simulink model "ArbBt"  (R2026a)
settings: Solver=FixedStepDiscrete  StopTime=10  FixedStep=0.005  EnableMultiTasking=on
undefined symbols (not defined in the file): absS, ArbBt_GradientInactive, ArbBt_GradientMax, ArbBt_GradientMin, ArbBt_PressureInactive, ArbBt_PressureMax, ArbBt_PressureMin, arbD, CLIP_HIGH_G, CLIP_HIGH_P, CLIP_LOW_G, CLIP_LOW_P, hps, ibBhms, PBP_CycleIndexTable, PBP_MAX_PROFILES, PBP_ProfileLength, PBP_ProfileStart, PBP_ProfileTable, PBP_SafeRow, PBP_StateType, ssm, tc, ysc
libraries: simulink x1
(part 1 of 2)
settings Model: DataDictionary=ArbBt_DataDictionary.sldd  Creator=72878  LastModifiedBy=72878
settings OptimizationCC: UseDivisionForNetSlopeComputation=on  DefaultUnderspecifiedDataType=single  InlineInvariantSignals=on  EfficientFloat2IntCast=on
settings DebuggingCC: SignalInfNanChecking=error  SignalRangeChecking=error  ReadBeforeWriteMsg=EnableAllAsWarning  WriteAfterWriteMsg=EnableAllAsWarning  WriteAfterReadMsg=EnableAllAsWarning  AlgebraicLoopMsg=error  ArtificialAlgebraicLoopMsg=error  SaveWithDisabledLinksMsg=error  SaveWithParameterizedLinksMsg=error  BlockPriorityViolationMsg=error  SolverPrmCheckMsg=error  InheritedTsInSrcMsg=error  MultiTaskRateTransMsg=warning  TasksWithSamePriorityMsg=error  SigSpecEnsureSampleTimeMsg=error  CheckMatrixSingularityMsg=error  IntegerOverflowMsg=error  ParameterUnderflowMsg=error  ParameterPrecisionLossMsg=error  UnderSpecifiedDataTypeMsg=error  UnnecessaryDatatypeConvMsg=warning  VectorMatrixConversionMsg=error  SignalLabelMismatchMsg=error  UnconnectedInputMsg=error  UnconnectedOutputMsg=error  UnconnectedLineMsg=error  SFcnCompatibilityMsg=error  BusObjectLabelMismatch=error  RootOutportRequireBusObject=error  AssertControl=DisableAll  ModelReferenceIOMismatchMessage=error  UnknownTsInhSupMsg=error  ModelReferenceDataLoggingMessage=error  StrictBusMsg=ErrorOnBusTreatedAsVector  NonBusSignalsTreatedAsBus=error  SFInvalidInputDataAccessInChartInitDiag=error  SFTransitionOutsideNaturalParentDiag=error  SFUnreachableExecutionPathDiag=error  SFUndirectedBroadcastEventsDiag=error  SFTransitionActionBeforeConditionDiag=error  SFTemporalDelaySmallerThanSampleTimeDiag=error  SFSelfTransitionDiag=error  SFExecutionAtInitializationDiag=error  IntegerSaturationMsg=error  VariantConditionMismatch=warning
settings SFSimCC: CompileTimeRecursionLimit=0.0  EnableRuntimeRecursion=off
settings RTWCC: SystemTargetFile=ert.tlc  EmbeddedCoderDictionary=ArbBt_DataDictionary.sldd  CustomHeaderCode="#include \"PBP_Config.h\""  CustomInclude="\"F:\\Onedrive_GN\\OneDrive - Brakes India Private Limited\\72878\\Nandini\\Electronic Stability Control\\POC\\MATLAB Models\\ARB_BT-PBP\\config\""  Description=Embedded Coder
settings CodeAppCC: IgnoreTestpoints=on  MATLABFcnDesc=on  MangleLength=4.0  MATLABSourceComments=on  ReqsInCode=on
settings ERTTargetCC: PreserveExpressionOrder=on  EnableSignedLeftShifts=off  EnableSignedRightShifts=off  UtilityFuncGeneration=Shared location  GenerateSampleERTMain=on  IncludeMdlTerminateFcn=off  SuppressErrorStatus=on  SupportNonFinite=off  ParenthesesLevel=Standards  CastingMode=Standards  GenerateSharedConstants=off
settings ConfigComp: CovScope=ReferencedModels  CovIncludeTopModel=off  CovForceBlockReductionOff=off

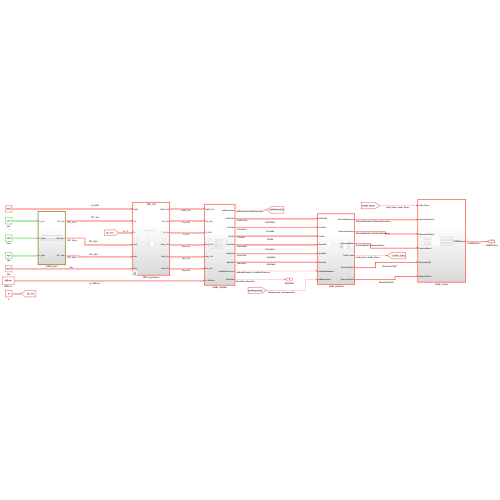
[thumbnail: Simulink's stored preview of the top-level diagram]
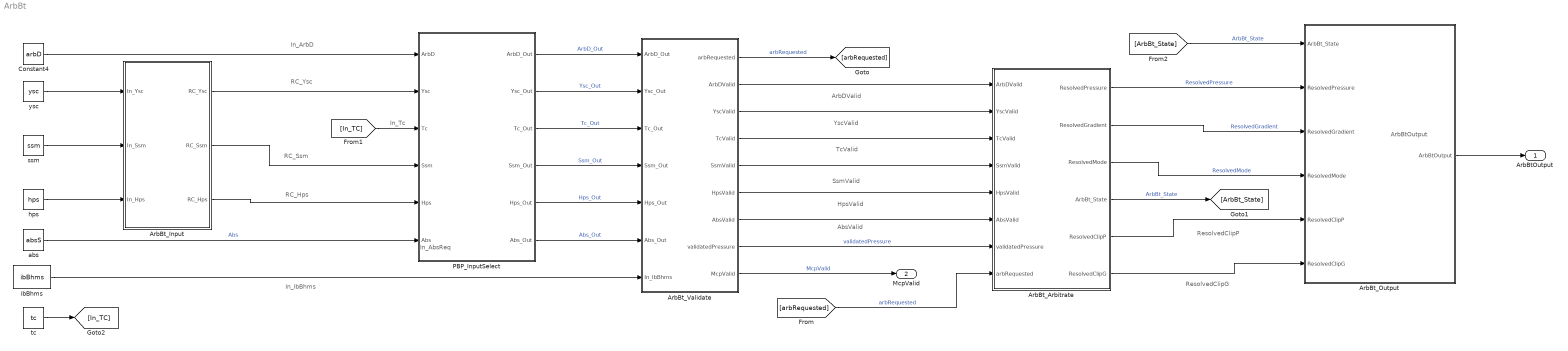
== system ArbBt ==
  note: SsmValid
  note: YscValid
  note: RC_Hps
  note: RC_Ssm
  note: RC_Ysc
  note: ArbBtOutput
  note: ArbDValid
  note: TcValid
  note: HpsValid
  note: AbsValid
  note: In_ArbD
  note: In_IbBhms
  note: In_AbsReq
  note: In_Tc
  note: ResolvedClipP
  note: ResolvedClipG
  ArbBt_Arbitrate : Subsystem  TreatAsAtomicUnit=on
  ArbBt_Input : Subsystem  TreatAsAtomicUnit=on
  ArbBt_Output : Subsystem  TreatAsAtomicUnit=on
  ArbBt_Validate : Subsystem  TreatAsAtomicUnit=on
  Constant4 : Constant  Value=arbD  OutDataTypeStr=Bus: Bus_ArbD  SampleTime=.005
  PBP_InputSelect : Subsystem  Variant=on  VariantActivationTime=code compile
  abs : Constant  Value=absS  OutDataTypeStr=Bus: Bus_Abs  SampleTime=.005
  hps : Constant  Value=hps  OutDataTypeStr=Bus: Bus_VcRequest  SampleTime=.01
  ibBhms : Constant  Value=ibBhms  OutDataTypeStr=Bus: Bus_IbBhms  SampleTime=.005
  ssm : Constant  Value=ssm  OutDataTypeStr=Bus: Bus_VcRequest  SampleTime=.01
  tc : Constant  Value=tc  OutDataTypeStr=Bus: Bus_VcRequest  SampleTime=.005
  ysc : Constant  Value=ysc  OutDataTypeStr=Bus: Bus_VcRequest  SampleTime=.01
  ArbBtOutput : Outport  OutDataTypeStr=Bus: Bus_Output  PortDimensions=1
  McpValid : Outport  Port=2  OutMin=0  OutMax=1  OutDataTypeStr=boolean  PortDimensions=1  SampleTime=0.005
  wires:
  ArbBt_Validate/2(ArbDValid) -> ArbBt_Arbitrate/1(ArbDValid)
  ArbBt_Validate/1(arbRequested) -> [arbRequested]  "arbRequested"
  ArbBt_Validate/8(validatedPressure) -> ArbBt_Arbitrate/7(validatedPressure)  "validatedPressure"
  ArbBt_Validate/6(HpsValid) -> ArbBt_Arbitrate/5(HpsValid)
  ArbBt_Validate/5(SsmValid) -> ArbBt_Arbitrate/4(SsmValid)
  ArbBt_Validate/4(TcValid) -> ArbBt_Arbitrate/3(TcValid)
  ArbBt_Validate/3(YscValid) -> ArbBt_Arbitrate/2(YscValid)
  [arbRequested] -> ArbBt_Arbitrate/8(arbRequested)  "arbRequested"
  ArbBt_Validate/9(McpValid) -> McpValid/1  "McpValid"
  ArbBt_Arbitrate/2(ResolvedGradient) -> ArbBt_Output/3(ResolvedGradient)  "ResolvedGradient"
  ArbBt_Arbitrate/3(ResolvedMode) -> ArbBt_Output/4(ResolvedMode)  "ResolvedMode"
  ArbBt_Output/1(ArbBtOutput) -> ArbBtOutput/1
  ArbBt_Arbitrate/4(ArbBt_State) -> [ArbBt_State]  "ArbBt_State"
  [ArbBt_State] -> ArbBt_Output/1(ArbBt_State)  "ArbBt_State"
  ArbBt_Arbitrate/1(ResolvedPressure) -> ArbBt_Output/2(ResolvedPressure)  "ResolvedPressure"
  ArbBt_Validate/7(AbsValid) -> ArbBt_Arbitrate/6(AbsValid)
  ArbBt_Arbitrate/5(ResolvedClipP) -> ArbBt_Output/5(ResolvedClipP)
  ArbBt_Arbitrate/6(ResolvedClipG) -> ArbBt_Output/6(ResolvedClipG)
  PBP_InputSelect/1(ArbD_Out) -> ArbBt_Validate/1(ArbD_Out)  "ArbD_Out"
  ArbBt_Input/1(RC_Ysc) -> PBP_InputSelect/2(Ysc)
  [In_TC] -> PBP_InputSelect/3(Tc)
  PBP_InputSelect/2(Ysc_Out) -> ArbBt_Validate/2(Ysc_Out)  "Ysc_Out"
  PBP_InputSelect/3(Tc_Out) -> ArbBt_Validate/3(Tc_Out)  "Tc_Out"
  PBP_InputSelect/4(Ssm_Out) -> ArbBt_Validate/4(Ssm_Out)  "Ssm_Out"
  PBP_InputSelect/5(Hps_Out) -> ArbBt_Validate/5(Hps_Out)  "Hps_Out"
  PBP_InputSelect/6(Abs_Out) -> ArbBt_Validate/6(Abs_Out)  "Abs_Out"
  ArbBt_Input/2(RC_Ssm) -> PBP_InputSelect/4(Ssm)
  ArbBt_Input/3(RC_Hps) -> PBP_InputSelect/5(Hps)
  ssm/1 -> ArbBt_Input/2(In_Ssm)
  ibBhms/1 -> ArbBt_Validate/7(In_IbBhms)
  Constant4/1 -> PBP_InputSelect/1(ArbD)
  hps/1 -> ArbBt_Input/3(In_Hps)
  tc/1 -> [In_TC]
  abs/1 -> PBP_InputSelect/6(Abs)  "Abs"
  ysc/1 -> ArbBt_Input/1(In_Ysc)

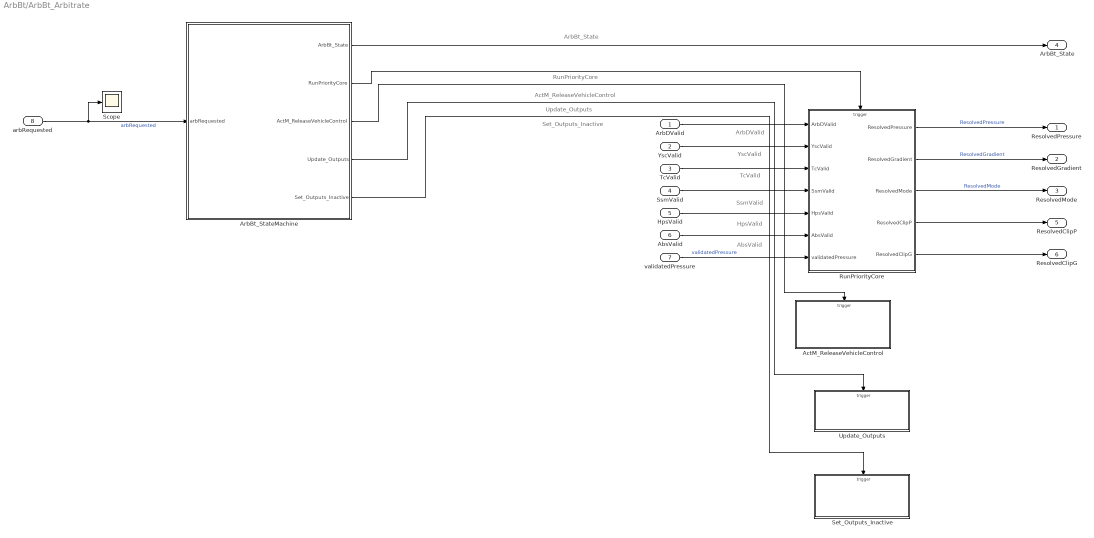
== system ArbBt/ArbBt_Arbitrate ==
  note: RunPriorityCore
  note: Set_Outputs_Inactive
  note: ActM_ReleaseVehicleControl
  note: AbsValid
  note: HpsValid
  note: SsmValid
  note: TcValid
  note: YscValid
  note: ArbDValid
  note: ArbBt_State
  note: Update_Outputs
  ArbDValid : Inport  OutDataTypeStr=Bus: ValidatedArbDBus  SampleTime=.005
  YscValid : Inport  Port=2  OutDataTypeStr=Bus: ValidatedVcRequestBus  SampleTime=.005
  TcValid : Inport  Port=3  OutDataTypeStr=Bus: ValidatedVcRequestBus  SampleTime=.005
  SsmValid : Inport  Port=4  OutDataTypeStr=Bus: ValidatedVcRequestBus  SampleTime=.005
  HpsValid : Inport  Port=5  OutDataTypeStr=Bus: ValidatedVcRequestBus  SampleTime=.005
  AbsValid : Inport  Port=6  OutDataTypeStr=Bus: ValidatedAbsBus  SampleTime=.005
  validatedPressure : Inport  Port=7  OutMin=0  OutMax=250  OutDataTypeStr=single  SampleTime=.005
  arbRequested : Inport  Port=8  OutMin=0  OutMax=1  OutDataTypeStr=boolean  SampleTime=0.005
  ActM_ReleaseVehicleControl : Subsystem
  ArbBt_StateMachine : Subsystem
  RunPriorityCore : Subsystem
  Scope : Scope
      settings: ActiveDisplayYMinimum=-1  ActiveDisplayYMaximum=1
  Set_Outputs_Inactive : Subsystem
  Update_Outputs : Subsystem
  ResolvedPressure : Outport  OutDataTypeStr=single
  ResolvedGradient : Outport  Port=2  OutDataTypeStr=single
  ResolvedMode : Outport  Port=3  OutDataTypeStr=Enum:ArbBtBrakeMode
  ArbBt_State : Outport  Port=4  OutDataTypeStr=Enum: ArbBtState
  ResolvedClipP : Outport  Port=5  OutDataTypeStr=boolean  PortDimensions=[1 4]
  ResolvedClipG : Outport  Port=6  OutDataTypeStr=boolean  PortDimensions=[1 4]
  wires:
  arbRequested/1 -> Scope/1, ArbBt_StateMachine/1(arbRequested)  "arbRequested"
  ArbDValid/1 -> RunPriorityCore/1(ArbDValid)
  YscValid/1 -> RunPriorityCore/2(YscValid)
  TcValid/1 -> RunPriorityCore/3(TcValid)
  SsmValid/1 -> RunPriorityCore/4(SsmValid)
  HpsValid/1 -> RunPriorityCore/5(HpsValid)
  AbsValid/1 -> RunPriorityCore/6(AbsValid)
  validatedPressure/1 -> RunPriorityCore/7(validatedPressure)  "validatedPressure"
  RunPriorityCore/1(ResolvedPressure) -> ResolvedPressure/1  "ResolvedPressure"
  RunPriorityCore/2(ResolvedGradient) -> ResolvedGradient/1  "ResolvedGradient"
  RunPriorityCore/3(ResolvedMode) -> ResolvedMode/1  "ResolvedMode"
  ArbBt_StateMachine/1(ArbBt_State) -> ArbBt_State/1
  ArbBt_StateMachine/2(RunPriorityCore) -> RunPriorityCore/Trigger
  ArbBt_StateMachine/4(Update_Outputs) -> Update_Outputs/Trigger
  ArbBt_StateMachine/5(Set_Outputs_Inactive) -> Set_Outputs_Inactive/Trigger
  RunPriorityCore/4(ResolvedClipP) -> ResolvedClipP/1
  RunPriorityCore/5(ResolvedClipG) -> ResolvedClipG/1
  ArbBt_StateMachine/3(ActM_ReleaseVehicleControl) -> ActM_ReleaseVehicleControl/Trigger

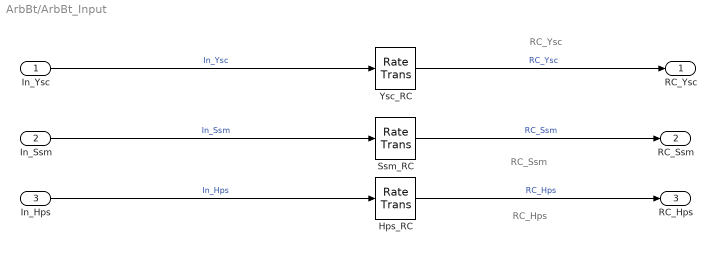
== system ArbBt/ArbBt_Input ==
  note: RC_Ysc
  note: RC_Ssm
  note: RC_Hps
  In_Ysc : Inport  OutDataTypeStr=Bus: Bus_VcRequest  SampleTime=.01
  In_Ssm : Inport  Port=2  OutDataTypeStr=Bus: Bus_VcRequest  SampleTime=.01
  In_Hps : Inport  Port=3  OutDataTypeStr=Bus: Bus_VcRequest  SampleTime=.01
  Hps_RC : RateTransition  OutPortSampleTime=0.005
  Ssm_RC : RateTransition  OutPortSampleTime=.005
  Ysc_RC : RateTransition  OutPortSampleTime=.005
  RC_Ysc : Outport  OutDataTypeStr=Bus: Bus_VcRequest  SampleTime=.005
  RC_Ssm : Outport  Port=2  OutDataTypeStr=Bus: Bus_VcRequest  SampleTime=0.005
  RC_Hps : Outport  Port=3  OutDataTypeStr=Bus: Bus_VcRequest  SampleTime=0.005
  wires:
  Ysc_RC/1 -> RC_Ysc/1  "RC_Ysc"
  Ssm_RC/1 -> RC_Ssm/1  "RC_Ssm"
  Hps_RC/1 -> RC_Hps/1  "RC_Hps"
  In_Ysc/1 -> Ysc_RC/1  "In_Ysc"
  In_Ssm/1 -> Ssm_RC/1  "In_Ssm"
  In_Hps/1 -> Hps_RC/1  "In_Hps"

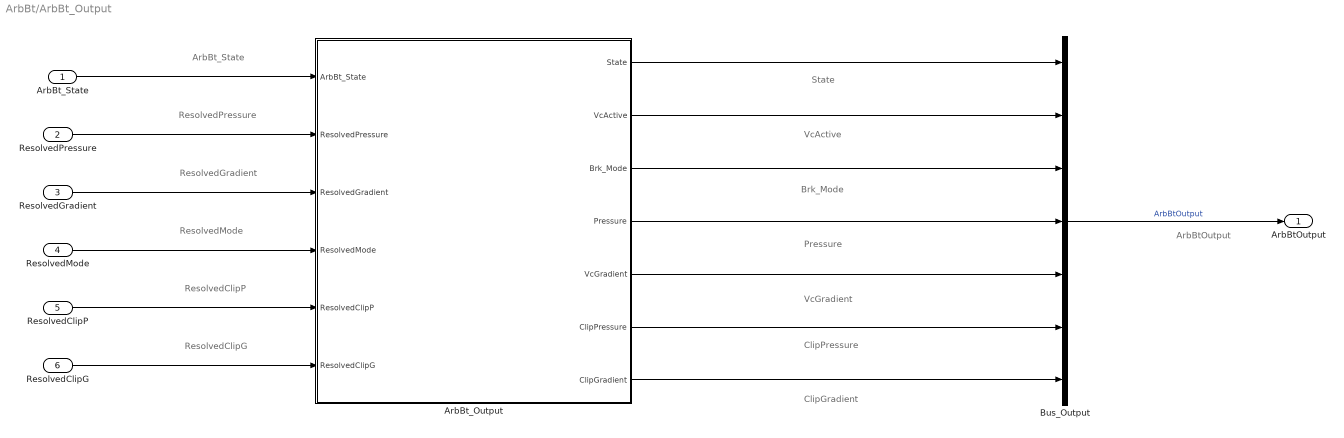
== system ArbBt/ArbBt_Output ==
  note: ResolvedClipP
  note: ArbBtOutput
  note: VcGradient
  note: Pressure
  note: Brk_Mode
  note: VcActive
  note: State
  note: ResolvedMode
  note: ResolvedGradient
  note: ResolvedPressure
  note: ArbBt_State
  note: ClipPressure
  note: ClipGradient
  note: ResolvedClipG
  ArbBt_State : Inport  OutDataTypeStr=Enum:ArbBtState
  ResolvedPressure : Inport  Port=2  OutDataTypeStr=single
  ResolvedGradient : Inport  Port=3  OutDataTypeStr=single
  ResolvedMode : Inport  Port=4  OutDataTypeStr=Enum:ArbBtBrakeMode
  ResolvedClipP : Inport  Port=5  OutDataTypeStr=boolean  PortDimensions=[1 4]
  ResolvedClipG : Inport  Port=6  OutDataTypeStr=boolean  PortDimensions=[1 4]
  ArbBt_Output : MATLAB Function  TreatAsAtomicUnit=on
  Bus_Output : BusCreator  Inputs=7  OutDataTypeStr=Bus: Bus_Output
  ArbBtOutput : Outport
  wires:
  ArbBt_State/1 -> ArbBt_Output/1(ArbBt_State)
  ResolvedPressure/1 -> ArbBt_Output/2(ResolvedPressure)
  ArbBt_Output/4(Pressure) -> Bus_Output/4
  ResolvedGradient/1 -> ArbBt_Output/3(ResolvedGradient)
  ResolvedMode/1 -> ArbBt_Output/4(ResolvedMode)
  ArbBt_Output/3(Brk_Mode) -> Bus_Output/3
  ArbBt_Output/1(State) -> Bus_Output/1
  ArbBt_Output/5(VcGradient) -> Bus_Output/5
  Bus_Output/1 -> ArbBtOutput/1  "ArbBtOutput"
  ArbBt_Output/2(VcActive) -> Bus_Output/2
  ResolvedClipP/1 -> ArbBt_Output/5(ResolvedClipP)
  ResolvedClipG/1 -> ArbBt_Output/6(ResolvedClipG)
  ArbBt_Output/6(ClipPressure) -> Bus_Output/6
  ArbBt_Output/7(ClipGradient) -> Bus_Output/7

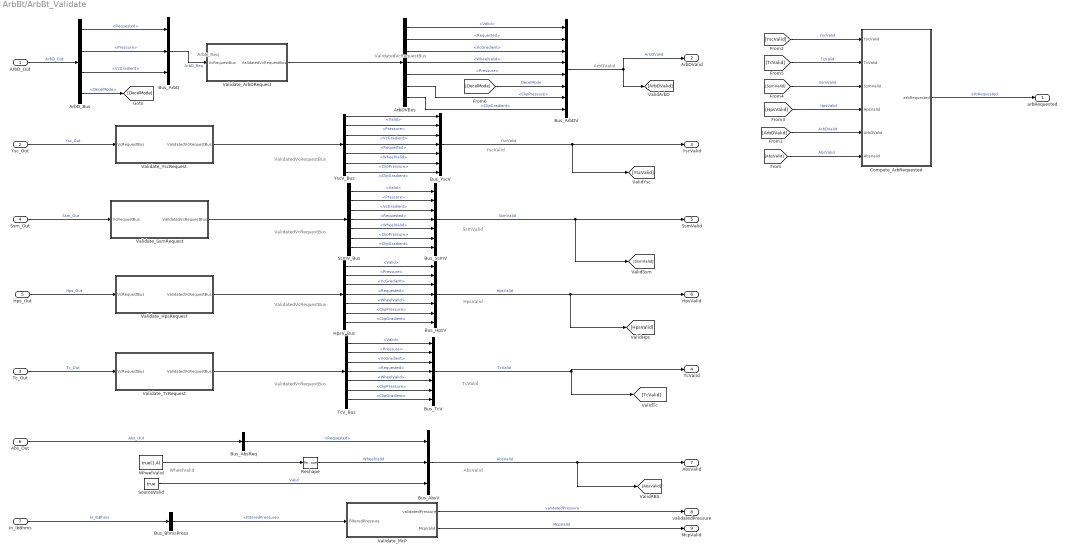
== system ArbBt/ArbBt_Validate ==
  note: HpsValid
  note: SsmValid
  note: TcValid
  note: YscValid
  note: ArbDValid
  note: ValidatedVcRequestBus
  note: ValidatedVcRequestBus
  note: ValidatedVcRequestBus
  note: ValidatedVcRequestBus
  note: ValidatedVcRequestBus
  note: ArbD_Req
  note: WheelValid
  note: AbsValid
  ArbD_Out : Inport  OutDataTypeStr=Bus: Bus_ArbD  SampleTime=0.005
  Ysc_Out : Inport  Port=2  OutDataTypeStr=Bus: Bus_VcRequest  SampleTime=0.005
  Tc_Out : Inport  Port=3  OutDataTypeStr=Bus: Bus_VcRequest  SampleTime=0.005
  Ssm_Out : Inport  Port=4  OutDataTypeStr=Bus: Bus_VcRequest  SampleTime=0.005
  Hps_Out : Inport  Port=5  OutDataTypeStr=Bus: Bus_VcRequest  SampleTime=0.005
  Abs_Out : Inport  Port=6  OutDataTypeStr=Bus: Bus_Abs  SampleTime=0.005
  In_IbBhms : Inport  Port=7  OutDataTypeStr=Bus: Bus_IbBhms  SampleTime=0.005
  ArbDVBus : BusSelector  OutputSignals=Valid,Requested,VcGradient,WheelValid,Pressure,ClipPressure,ClipGradient
  ArbD_Bus : BusSelector  OutputSignals=Requested,Pressure,VcGradient,DecelMode
  Bus_AbsReq : BusSelector  OutputSignals=Requested
  Bus_AbsV : BusCreator  Inputs=3  OutDataTypeStr=Bus: ValidatedAbsBus
      settings: InheritFromInputs=off
  Bus_ArbD : BusCreator  Inputs=3  OutDataTypeStr=Bus: Bus_VcRequest
  Bus_ArbDV : BusCreator  Inputs=8  OutDataTypeStr=Bus: ValidatedArbDBus
  Bus_BhmsPress : BusSelector  OutputSignals=FilteredPressure
  Bus_HpsV : BusCreator  Inputs=7
  Bus_SsmV : BusCreator  Inputs=7
  Bus_TcV : BusCreator  Inputs=7
  Bus_YscV : BusCreator  Inputs=7
  Compute_ArbRequested : MATLAB Function  TreatAsAtomicUnit=on
  HpsV_Bus : BusSelector  OutputSignals=Valid,Pressure,VcGradient,Requested,WheelValid,ClipPressure,ClipGradient
  Reshape : Reshape  OutputDimensionality=Row vector (2-D)
  SourceValid : Constant  Value=true  OutDataTypeStr=boolean  SampleTime=.005
  SsmV_Bus : BusSelector  OutputSignals=Valid,Pressure,VcGradient,Requested,WheelValid,ClipPressure,ClipGradient
  TcV_Bus : BusSelector  OutputSignals=Valid,Pressure,VcGradient,Requested,WheelValid,ClipPressure,ClipGradient
  Validate_ArbDRequest : MATLAB Function  TreatAsAtomicUnit=on
  Validate_HpsRequest : MATLAB Function  TreatAsAtomicUnit=on
  Validate_McP : MATLAB Function  TreatAsAtomicUnit=on
  Validate_SsmRequest : MATLAB Function  TreatAsAtomicUnit=on
  Validate_TcRequest : MATLAB Function  TreatAsAtomicUnit=on
  Validate_YscRequest : MATLAB Function  TreatAsAtomicUnit=on
  WheelValid : Constant  Value=true(1,4)  OutDataTypeStr=boolean  SampleTime=.005
  YscV_Bus : BusSelector  OutputSignals=Valid,Pressure,VcGradient,Requested,WheelValid,ClipPressure,ClipGradient
  arbRequested : Outport  OutMin=0  OutMax=1  OutDataTypeStr=boolean  PortDimensions=1  SampleTime=.005
  ArbDValid : Outport  Port=2  OutDataTypeStr=Bus: ValidatedArbDBus  SampleTime=0.005
  YscValid : Outport  Port=3  OutDataTypeStr=Bus: ValidatedVcRequestBus  SampleTime=0.005
  TcValid : Outport  Port=4  OutDataTypeStr=Bus: ValidatedVcRequestBus  SampleTime=0.005
  SsmValid : Outport  Port=5  OutDataTypeStr=Bus: ValidatedVcRequestBus  SampleTime=.005
  HpsValid : Outport  Port=6  OutDataTypeStr=Bus: ValidatedVcRequestBus  SampleTime=0.005
  AbsValid : Outport  Port=7  OutDataTypeStr=Bus: ValidatedAbsBus  SampleTime=0.005
  validatedPressure : Outport  Port=8  OutMin=0  OutMax=250  OutDataTypeStr=single  Unit=bar
  McpValid : Outport  Port=9  OutMin=0  OutMax=1  OutDataTypeStr=boolean
  wires:
  Ysc_Out/1 -> Validate_YscRequest/1(VcRequestBus)  "Ysc_Out"
  Tc_Out/1 -> Validate_TcRequest/1(VcRequestBus)  "Tc_Out"
  Ssm_Out/1 -> Validate_SsmRequest/1(VcRequestBus)  "Ssm_Out"
  ArbD_Out/1 -> ArbD_Bus/1  "ArbD_Out"
  ArbD_Bus/1 -> Bus_ArbD/1  "<Requested>"
  Bus_ArbD/1 -> Validate_ArbDRequest/1(VcRequestBus)  "ArbD_Req"
  Validate_YscRequest/1(ValidatedVcRequestBus) -> YscV_Bus/1
  YscV_Bus/1 -> Bus_YscV/1  "<Valid>"
  YscV_Bus/2 -> Bus_YscV/2  "<Pressure>"
  YscV_Bus/3 -> Bus_YscV/3  "<VcGradient>"
  YscV_Bus/4 -> Bus_YscV/4  "<Requested>"
  YscV_Bus/5 -> Bus_YscV/5  "<WheelValid>"
  TcV_Bus/3 -> Bus_TcV/3  "<VcGradient>"
  Validate_TcRequest/1(ValidatedVcRequestBus) -> TcV_Bus/1
  TcV_Bus/1 -> Bus_TcV/1  "<Valid>"
  TcV_Bus/4 -> Bus_TcV/4  "<Requested>"
  TcV_Bus/2 -> Bus_TcV/2  "<Pressure>"
  TcV_Bus/5 -> Bus_TcV/5  "<WheelValid>"
  SsmV_Bus/5 -> Bus_SsmV/5  "<WheelValid>"
  Validate_SsmRequest/1(ValidatedVcRequestBus) -> SsmV_Bus/1
  SsmV_Bus/1 -> Bus_SsmV/1  "<Valid>"
  SsmV_Bus/2 -> Bus_SsmV/2  "<Pressure>"
  SsmV_Bus/4 -> Bus_SsmV/4  "<Requested>"
  SsmV_Bus/3 -> Bus_SsmV/3  "<VcGradient>"
  HpsV_Bus/1 -> Bus_HpsV/1  "<Valid>"
  HpsV_Bus/2 -> Bus_HpsV/2  "<Pressure>"
  HpsV_Bus/5 -> Bus_HpsV/5  "<WheelValid>"
  HpsV_Bus/4 -> Bus_HpsV/4  "<Requested>"
  Validate_HpsRequest/1(ValidatedVcRequestBus) -> HpsV_Bus/1
  Validate_ArbDRequest/1(ValidatedVcRequestBus) -> ArbDVBus/1
  ArbDVBus/1 -> Bus_ArbDV/1  "<Valid>"
  ArbDVBus/2 -> Bus_ArbDV/2  "<Requested>"
  ArbDVBus/4 -> Bus_ArbDV/4  "<WheelValid>"
  ArbDVBus/5 -> Bus_ArbDV/5  "<Pressure>"
  SourceValid/1 -> Bus_AbsV/3  "Valid"
  [ArbDValid] -> Compute_ArbRequested/5(ArbDValid)  "ArbDValid"
  [YscValid] -> Compute_ArbRequested/1(YscValid)  "YscValid"
  [TcValid] -> Compute_ArbRequested/2(TcValid)  "TcValid"
  [SsmValid] -> Compute_ArbRequested/3(SsmValid)  "SsmValid"
  [HpsValid] -> Compute_ArbRequested/4(HpsValid)  "HpsValid"
  [AbsValid] -> Compute_ArbRequested/6(AbsValid)  "AbsValid"
  Compute_ArbRequested/1(arbRequested) -> arbRequested/1  "arbRequested"
  Validate_McP/1(validatedPressure) -> validatedPressure/1  "validatedPressure"
  Validate_McP/2(McpValid) -> McpValid/1  "McpValid"
  Bus_ArbDV/1 -> [ArbDValid], ArbDValid/1  "ArbDValid"
  Bus_YscV/1 -> YscValid/1, [YscValid]  "YscValid"
  Bus_TcV/1 -> TcValid/1, [TcValid]  "TcValid"
  Bus_SsmV/1 -> [SsmValid], SsmValid/1  "SsmValid"
  Bus_HpsV/1 -> [HpsValid], HpsValid/1  "HpsValid"
  Bus_AbsV/1 -> AbsValid/1, [AbsValid]  "AbsValid"
  Abs_Out/1 -> Bus_AbsReq/1  "Abs_Out"
  Bus_AbsReq/1 -> Bus_AbsV/1  "<Requested>"
  ArbD_Bus/2 -> Bus_ArbD/2  "<Pressure>"
  [DecelMode] -> Bus_ArbDV/6  "DecelMode"
  ArbDVBus/3 -> Bus_ArbDV/3  "<VcGradient>"
  HpsV_Bus/3 -> Bus_HpsV/3  "<VcGradient>"
  ArbD_Bus/3 -> Bus_ArbD/3  "<VcGradient>"
  ArbD_Bus/4 -> [DecelMode]  "<DecelMode>"
  WheelValid/1 -> Reshape/1
  Reshape/1 -> Bus_AbsV/2  "WheelValid"
  Bus_BhmsPress/1 -> Validate_McP/1(FilteredPressure)  "<FilteredPressure>"
  In_IbBhms/1 -> Bus_BhmsPress/1  "In_IbBhms"
  Hps_Out/1 -> Validate_HpsRequest/1(VcRequestBus)  "Hps_Out"
  ArbDVBus/6 -> Bus_ArbDV/7  "<ClipPressure>"
  ArbDVBus/7 -> Bus_ArbDV/8  "<ClipGradient>"
  YscV_Bus/6 -> Bus_YscV/6  "<ClipPressure>"
  YscV_Bus/7 -> Bus_YscV/7  "<ClipGradient>"
  SsmV_Bus/6 -> Bus_SsmV/6  "<ClipPressure>"
  SsmV_Bus/7 -> Bus_SsmV/7  "<ClipGradient>"
  HpsV_Bus/6 -> Bus_HpsV/6  "<ClipPressure>"
  HpsV_Bus/7 -> Bus_HpsV/7  "<ClipGradient>"
  TcV_Bus/6 -> Bus_TcV/6  "<ClipPressure>"
  TcV_Bus/7 -> Bus_TcV/7  "<ClipGradient>"

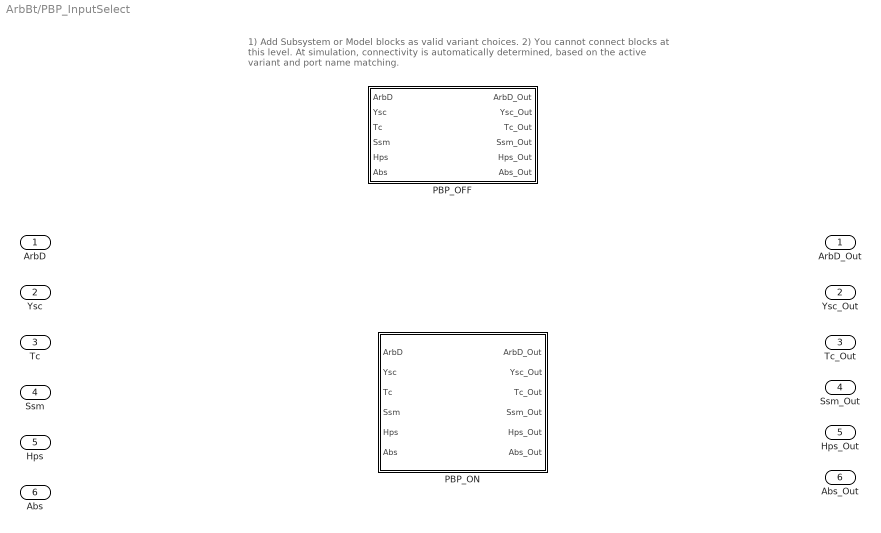
== system ArbBt/PBP_InputSelect ==
  note: 1) Add Subsystem or Model blocks as valid variant choices.
      | 2) You cannot connect blocks at this level. At simulation, connectivity is automatically
      | determined, based on the active variant and port name matching.
  ArbD : Inport
  Ysc : Inport  Port=2
  Tc : Inport  Port=3
  Ssm : Inport  Port=4
  Hps : Inport  Port=5
  Abs : Inport  Port=6
  PBP_OFF : Subsystem  TreatAsAtomicUnit=on  VariantControl=Enable_PBP_Test_Interface ==0
      settings: RTWSystemCode=Inline
  PBP_ON : Subsystem  TreatAsAtomicUnit=on  VariantControl=Enable_PBP_Test_Interface ==1
      settings: RTWSystemCode=Inline
  ArbD_Out : Outport
  Ysc_Out : Outport  Port=2
  Tc_Out : Outport  Port=3
  Ssm_Out : Outport  Port=4
  Hps_Out : Outport  Port=5
  Abs_Out : Outport  Port=6

== system ArbBt/ArbBt_Arbitrate/ActM_ReleaseVehicleControl ==
  ActM_ReleaseVehicleControl : TriggerPort  TriggerType=function-call  VariantControl=(inherit)
  ReleaseWrapper : Subsystem  Variant=on  VariantActivationTime=code compile

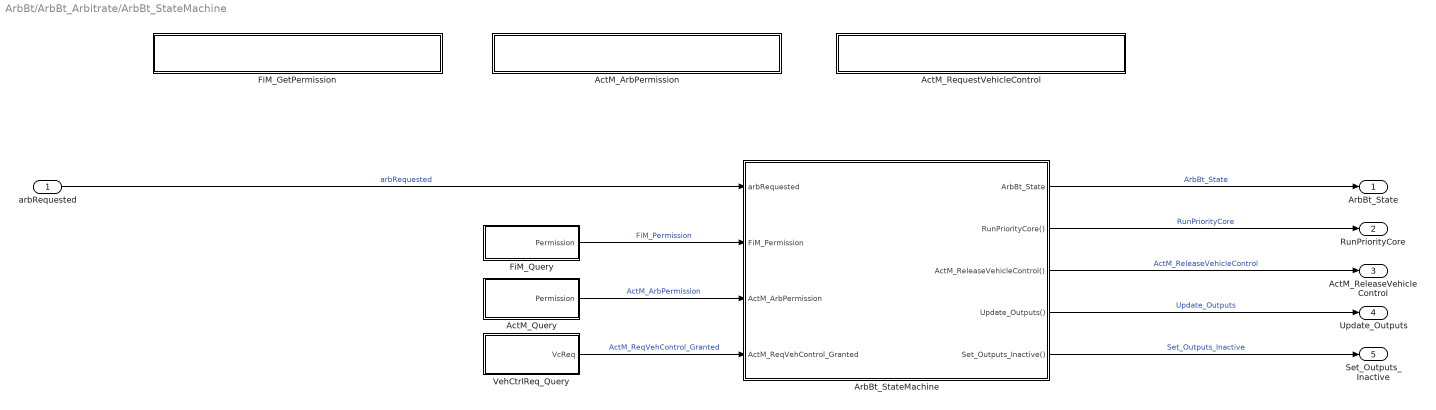
== system ArbBt/ArbBt_Arbitrate/ArbBt_StateMachine ==
  arbRequested : Inport  OutDataTypeStr=boolean
  ActM_ArbPermission : Subsystem  TreatAsAtomicUnit=on
  ActM_Query : Subsystem  Variant=on  VariantActivationTime=code compile
  ActM_RequestVehicleControl : Subsystem  TreatAsAtomicUnit=on
  ArbBt_StateMachine : Stateflow chart  TreatAsAtomicUnit=on
  FiM_GetPermission : Subsystem  TreatAsAtomicUnit=on
  FiM_Query : Subsystem  Variant=on  VariantActivationTime=code compile
  VehCtrlReq_Query : Subsystem  Variant=on  VariantActivationTime=code compile
  ArbBt_State : Outport  OutDataTypeStr=Enum: ArbBtState
  RunPriorityCore : Outport  Port=2
  ActM_ReleaseVehicleControl : Outport  Port=3
  Update_Outputs : Outport  Port=4
  Set_Outputs_Inactive : Outport  Port=5
  wires:
  FiM_Query/1(Permission) -> ArbBt_StateMachine/2(FiM_Permission)  "FiM_Permission"
  arbRequested/1 -> ArbBt_StateMachine/1(arbRequested)  "arbRequested"
  VehCtrlReq_Query/1(VcReq) -> ArbBt_StateMachine/4(ActM_ReqVehControl_Granted)  "ActM_ReqVehControl_Granted"
  ArbBt_StateMachine/2(RunPriorityCore()) -> RunPriorityCore/1  "RunPriorityCore"
  ArbBt_StateMachine/3(ActM_ReleaseVehicleControl()) -> ActM_ReleaseVehicleControl/1  "ActM_ReleaseVehicleControl"
  ArbBt_StateMachine/4(Update_Outputs()) -> Update_Outputs/1  "Update_Outputs"
  ArbBt_StateMachine/5(Set_Outputs_Inactive()) -> Set_Outputs_Inactive/1  "Set_Outputs_Inactive"
  ArbBt_StateMachine/1(ArbBt_State) -> ArbBt_State/1  "ArbBt_State"
  ActM_Query/1(Permission) -> ArbBt_StateMachine/3(ActM_ArbPermission)  "ActM_ArbPermission"

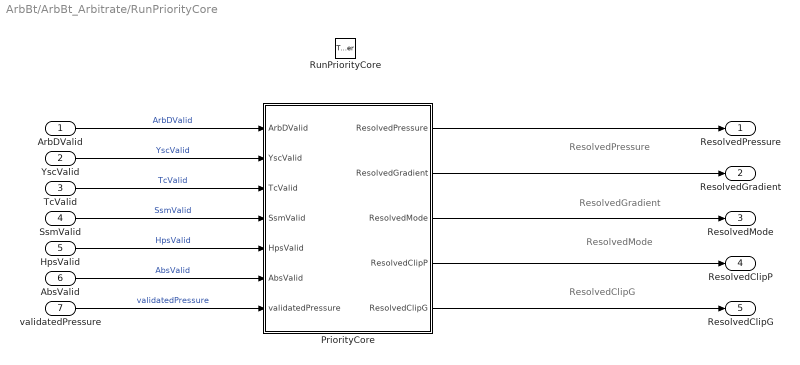
== system ArbBt/ArbBt_Arbitrate/RunPriorityCore ==
  note: ResolvedMode
  note: ResolvedGradient
  note: ResolvedPressure
  note: ResolvedClipG
  ArbDValid : Inport
  YscValid : Inport  Port=2
  TcValid : Inport  Port=3
  SsmValid : Inport  Port=4
  HpsValid : Inport  Port=5
  AbsValid : Inport  Port=6
  validatedPressure : Inport  Port=7  OutDataTypeStr=single
  RunPriorityCore : TriggerPort  TriggerType=function-call  VariantControl=(inherit)
  PriorityCore : Subsystem
  ResolvedPressure : Outport
  ResolvedGradient : Outport  Port=2
  ResolvedMode : Outport  Port=3
  ResolvedClipP : Outport  Port=4
  ResolvedClipG : Outport  Port=5
  wires:
  AbsValid/1 -> PriorityCore/6(AbsValid)  "AbsValid"
  ArbDValid/1 -> PriorityCore/1(ArbDValid)  "ArbDValid"
  validatedPressure/1 -> PriorityCore/7(validatedPressure)  "validatedPressure"
  YscValid/1 -> PriorityCore/2(YscValid)  "YscValid"
  SsmValid/1 -> PriorityCore/4(SsmValid)  "SsmValid"
  HpsValid/1 -> PriorityCore/5(HpsValid)  "HpsValid"
  TcValid/1 -> PriorityCore/3(TcValid)  "TcValid"
  PriorityCore/1(ResolvedPressure) -> ResolvedPressure/1
  PriorityCore/2(ResolvedGradient) -> ResolvedGradient/1
  PriorityCore/3(ResolvedMode) -> ResolvedMode/1
  PriorityCore/4(ResolvedClipP) -> ResolvedClipP/1
  PriorityCore/5(ResolvedClipG) -> ResolvedClipG/1

== system ArbBt/ArbBt_Arbitrate/Set_Outputs_Inactive ==
  Set_Outputs_Inactive : TriggerPort  TriggerType=function-call  VariantControl=(inherit)
  SetOutputsInactive : MATLAB Function  TreatAsAtomicUnit=on

== system ArbBt/ArbBt_Arbitrate/Update_Outputs ==
  Update_Outputs : TriggerPort  TriggerType=function-call  VariantControl=(inherit)
  Update_out : MATLAB Function  TreatAsAtomicUnit=on

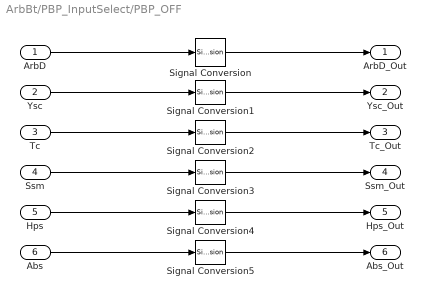
== system ArbBt/PBP_InputSelect/PBP_OFF ==
  ArbD : Inport  OutDataTypeStr=Bus: Bus_ArbD  SampleTime=.005
  Ysc : Inport  Port=2  OutDataTypeStr=Bus: Bus_VcRequest  SampleTime=.005
  Tc : Inport  Port=3  OutDataTypeStr=Bus: Bus_VcRequest  SampleTime=.005
  Ssm : Inport  Port=4  OutDataTypeStr=Bus: Bus_VcRequest  SampleTime=.005
  Hps : Inport  Port=5  OutDataTypeStr=Bus: Bus_VcRequest  SampleTime=.005
  Abs : Inport  Port=6  OutDataTypeStr=Bus: Bus_Abs  SampleTime=.005
  Signal Conversion : SignalConversion  ConversionOutput=Nonvirtual bus  OutDataTypeStr=Bus: Bus_ArbD  OverrideOpt=off
  Signal Conversion{1..4} (4 alike) : SignalConversion  ConversionOutput=Nonvirtual bus  OutDataTypeStr=Bus: Bus_VcRequest  OverrideOpt=off
  Signal Conversion5 : SignalConversion  ConversionOutput=Nonvirtual bus  OutDataTypeStr=Bus: Bus_Abs  OverrideOpt=off
  ArbD_Out : Outport  OutDataTypeStr=Bus: Bus_ArbD
  Ysc_Out : Outport  Port=2  OutDataTypeStr=Bus: Bus_VcRequest  SampleTime=.005
  Tc_Out : Outport  Port=3  OutDataTypeStr=Bus: Bus_VcRequest
  Ssm_Out : Outport  Port=4  OutDataTypeStr=Bus: Bus_VcRequest  SampleTime=.005
  Hps_Out : Outport  Port=5  OutDataTypeStr=Bus: Bus_VcRequest
  Abs_Out : Outport  Port=6  OutDataTypeStr=Bus: Bus_Abs
  wires:
  Abs/1 -> Signal Conversion5/1
  Hps/1 -> Signal Conversion4/1
  Tc/1 -> Signal Conversion2/1
  Ysc/1 -> Signal Conversion1/1
  ArbD/1 -> Signal Conversion/1
  Ssm/1 -> Signal Conversion3/1
  Signal Conversion/1 -> ArbD_Out/1
  Signal Conversion1/1 -> Ysc_Out/1
  Signal Conversion2/1 -> Tc_Out/1
  Signal Conversion3/1 -> Ssm_Out/1
  Signal Conversion4/1 -> Hps_Out/1
  Signal Conversion5/1 -> Abs_Out/1

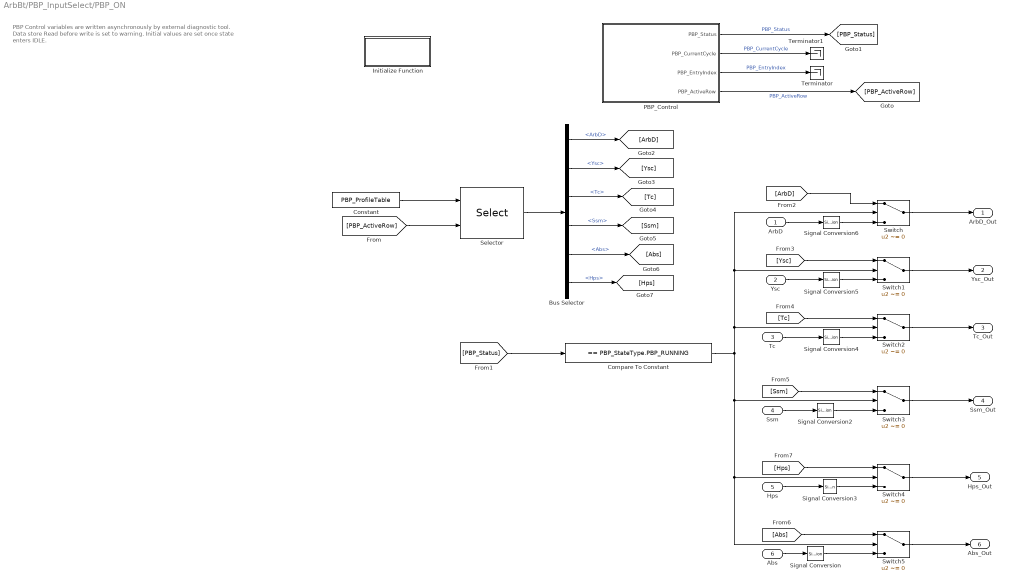
== system ArbBt/PBP_InputSelect/PBP_ON ==
  note: PBP Control variables are written asynchronously by external diagnostic tool.
      | Data store Read before write is set to warning. Initial values are set once state enters IDLE.
  ArbD : Inport  OutDataTypeStr=Bus: Bus_ArbD  SampleTime=.005
  Ysc : Inport  Port=2  OutDataTypeStr=Bus: Bus_VcRequest  SampleTime=.005
  Tc : Inport  Port=3  OutDataTypeStr=Bus: Bus_VcRequest  SampleTime=.005
  Ssm : Inport  Port=4  OutDataTypeStr=Bus: Bus_VcRequest  SampleTime=.005
  Hps : Inport  Port=5  OutDataTypeStr=Bus: Bus_VcRequest  SampleTime=.005
  Abs : Inport  Port=6  OutDataTypeStr=Bus: Bus_Abs  SampleTime=.005
  Bus Selector : BusSelector  OutputSignals=ArbD,Ysc,Tc,Ssm,Abs,Hps
  Compare To Constant : simulink/Logic and Bit Operations/Compare To Constant  relop===  const=PBP_StateType.PBP_RUNNING  OutDataTypeStr=boolean
  Constant : Constant  Value=PBP_ProfileTable  OutDataTypeStr=Bus: PBP_Entry_t  SampleTime=.005
  Initialize Function : Subsystem  TreatAsAtomicUnit=on
  PBP_Control : Subsystem  TreatAsAtomicUnit=on  RTWFileName=PBP
      settings: RTWSystemCode=Nonreusable function  RTWFileNameOpts=User specified
  Selector : Selector  IndexMode=Zero-based  IndexOptions=Index vector (port)  Indices=[1 3]  OutputSizes=1
  Signal Conversion : SignalConversion  ConversionOutput=Nonvirtual bus  OutDataTypeStr=Bus: Bus_Abs  OverrideOpt=off
  Signal Conversion{2..5} (4 alike) : SignalConversion  ConversionOutput=Nonvirtual bus  OutDataTypeStr=Bus: Bus_VcRequest  OverrideOpt=off
  Signal Conversion6 : SignalConversion  ConversionOutput=Nonvirtual bus  OutDataTypeStr=Bus: Bus_ArbD  OverrideOpt=off
  Switch{,1..5} (6 alike) : Switch  Criteria=u2 ~= 0  SaturateOnIntegerOverflow=off  InputSameDT=off
  Terminator : Terminator
  Terminator1 : Terminator
  ArbD_Out : Outport
  Ysc_Out : Outport  Port=2
  Tc_Out : Outport  Port=3
  Ssm_Out : Outport  Port=4
  Hps_Out : Outport  Port=5
  Abs_Out : Outport  Port=6
  wires:
  PBP_Control/3(PBP_EntryIndex) -> Terminator/1  "PBP_EntryIndex"
  PBP_Control/1(PBP_Status) -> [PBP_Status]  "PBP_Status"
  PBP_Control/2(PBP_CurrentCycle) -> Terminator1/1  "PBP_CurrentCycle"
  PBP_Control/4(PBP_ActiveRow) -> [PBP_ActiveRow]  "PBP_ActiveRow"
  ArbD/1 -> Signal Conversion6/1
  Tc/1 -> Signal Conversion4/1
  Ysc/1 -> Signal Conversion5/1
  Constant/1 -> Selector/1
  [PBP_ActiveRow] -> Selector/2
  Selector/1 -> Bus Selector/1
  Compare To Constant/1 -> Switch/2, Switch1/2, Switch2/2, Switch4/2, Switch5/2, Switch3/2
  [PBP_Status] -> Compare To Constant/1
  Switch/1 -> ArbD_Out/1
  Switch1/1 -> Ysc_Out/1
  Switch2/1 -> Tc_Out/1
  Switch3/1 -> Ssm_Out/1
  Switch4/1 -> Hps_Out/1
  Switch5/1 -> Abs_Out/1
  Bus Selector/1 -> [ArbD]  "<ArbD>"
  [ArbD] -> Switch/1
  Bus Selector/2 -> [Ysc]  "<Ysc>"
  [Ysc] -> Switch1/1
  Bus Selector/3 -> [Tc]  "<Tc>"
  [Tc] -> Switch2/1
  Bus Selector/4 -> [Ssm]  "<Ssm>"
  [Ssm] -> Switch3/1
  Bus Selector/5 -> [Abs]  "<Abs>"
  Bus Selector/6 -> [Hps]  "<Hps>"
  [Hps] -> Switch4/1
  [Abs] -> Switch5/1
  Abs/1 -> Signal Conversion/1
  Signal Conversion/1 -> Switch5/3
  Ssm/1 -> Signal Conversion2/1
  Signal Conversion2/1 -> Switch3/3
  Hps/1 -> Signal Conversion3/1
  Signal Conversion3/1 -> Switch4/3
  Signal Conversion4/1 -> Switch2/3
  Signal Conversion5/1 -> Switch1/3
  Signal Conversion6/1 -> Switch/3

== system ArbBt/ArbBt_Arbitrate/ActM_ReleaseVehicleControl/ReleaseWrapper ==
  note: 1) Add Subsystem or Model blocks as valid variant choices.
      | 2) You cannot connect blocks at this level. At simulation, connectivity is automatically
      | determined, based on the active variant and port name matching.
  PBP_OFF : Subsystem  TreatAsAtomicUnit=on  VariantControl=Enable_PBP_Test_Interface == 0
      settings: RTWSystemCode=Inline
  PBP_ON : Subsystem  TreatAsAtomicUnit=on  VariantControl=Enable_PBP_Test_Interface == 1
      settings: RTWSystemCode=Inline

== system ArbBt/ArbBt_Arbitrate/ArbBt_StateMachine/ActM_ArbPermission ==
  ActM_GetArbitratorPermission : TriggerPort  TriggerType=function-call  IsSimulinkFunction=on  FunctionName=ActM_GetArbitratorPermission  FunctionVisibility=scoped  VariantControl=(inherit)
  ActM_True : Constant  Value=true  OutDataTypeStr=boolean  SampleTime=-1
  ActM_permission : ArgOut  DisableCoverage=on  OutDataTypeStr=boolean  ArgumentName=ActM_ArbPermission
  wires:
  ActM_True/1 -> ActM_permission/1  "DefaultTruep_ActM"

== system ArbBt/ArbBt_Arbitrate/ArbBt_StateMachine/ActM_Query ==
  note: 1) Add Subsystem or Model blocks as valid variant choices.
      | 2) You cannot connect blocks at this level. At simulation, connectivity is automatically
      | determined, based on the active variant and port name matching.
  PBP_OFF : Subsystem  TreatAsAtomicUnit=on  VariantControl=Enable_PBP_Test_Interface == 0
      settings: RTWSystemCode=Inline
  PBP_ON : Subsystem  TreatAsAtomicUnit=on  VariantControl=Enable_PBP_Test_Interface == 1
      settings: RTWSystemCode=Inline
  Permission : Outport

== system ArbBt/ArbBt_Arbitrate/ArbBt_StateMachine/ActM_RequestVehicleControl ==
  ActM_RequestVehicleControl : TriggerPort  TriggerType=function-call  IsSimulinkFunction=on  FunctionName=ActM_RequestVehicleControl  FunctionVisibility=scoped  VariantControl=(inherit)
  VcReq_True : Constant  Value=true  OutDataTypeStr=boolean  SampleTime=-1
  ActM_ReqVehControl_Granted : ArgOut  DisableCoverage=on  OutDataTypeStr=boolean  ArgumentName=ActM_ReqVehControl_Granted
  wires:
  VcReq_True/1 -> ActM_ReqVehControl_Granted/1  "DefaultTrue_VcReq"

== system ArbBt/ArbBt_Arbitrate/ArbBt_StateMachine/FiM_GetPermission ==
  FiM_GetFunctionPermission : TriggerPort  TriggerType=function-call  IsSimulinkFunction=on  FunctionName=FiM_GetFunctionPermission  FunctionVisibility=scoped  VariantControl=(inherit)
  FiM_True : Constant  Value=true  OutDataTypeStr=boolean  SampleTime=-1
  FiM_permission : ArgOut  DisableCoverage=on  OutDataTypeStr=boolean  ArgumentName=FiM_permission
  wires:
  FiM_True/1 -> FiM_permission/1  "DefaultTrue_FiM"

== system ArbBt/ArbBt_Arbitrate/ArbBt_StateMachine/FiM_Query ==
  note: 1) Add Subsystem or Model blocks as valid variant choices.
      | 2) You cannot connect blocks at this level. At simulation, connectivity is automatically
      | determined, based on the active variant and port name matching.
  PBP_OFF : Subsystem  TreatAsAtomicUnit=on  VariantControl=Enable_PBP_Test_Interface == 0
      settings: RTWSystemCode=Inline
  PBP_ON : Subsystem  TreatAsAtomicUnit=on  VariantControl=Enable_PBP_Test_Interface == 1
      settings: RTWSystemCode=Inline
  Permission : Outport

== system ArbBt/ArbBt_Arbitrate/ArbBt_StateMachine/VehCtrlReq_Query ==
  note: 1) Add Subsystem or Model blocks as valid variant choices.
      | 2) You cannot connect blocks at this level. At simulation, connectivity is automatically
      | determined, based on the active variant and port name matching.
  PBP_OFF : Subsystem  TreatAsAtomicUnit=on  VariantControl=Enable_PBP_Test_Interface == 0
      settings: RTWSystemCode=Inline
  PBP_ON : Subsystem  TreatAsAtomicUnit=on  VariantControl=Enable_PBP_Test_Interface == 1
      settings: RTWSystemCode=Inline
  VcReq : Outport

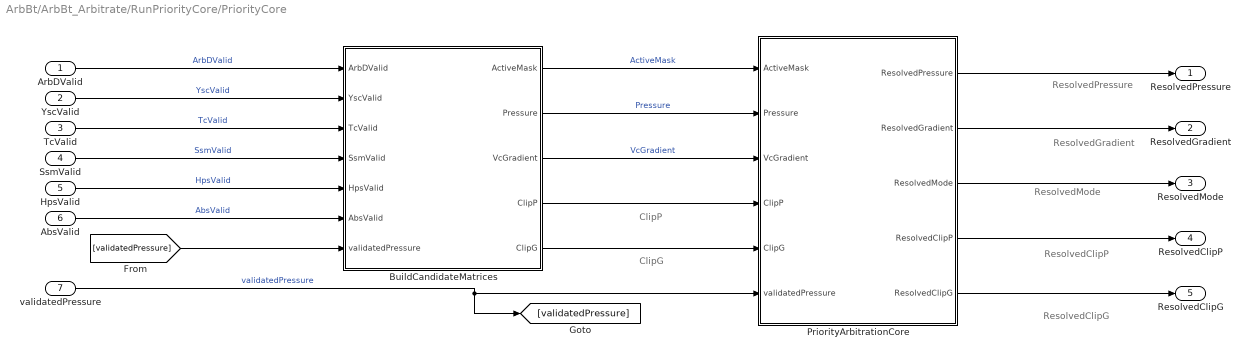
== system ArbBt/ArbBt_Arbitrate/RunPriorityCore/PriorityCore ==
  note: ResolvedMode
  note: ResolvedGradient
  note: ResolvedPressure
  note: ResolvedClipP
  note: ResolvedClipG
  note: ClipP
  note: ClipG
  ArbDValid : Inport
  YscValid : Inport  Port=2
  TcValid : Inport  Port=3
  SsmValid : Inport  Port=4
  HpsValid : Inport  Port=5
  AbsValid : Inport  Port=6
  validatedPressure : Inport  Port=7  OutMax=250  OutDataTypeStr=single  Unit=bar
  BuildCandidateMatrices : MATLAB Function  TreatAsAtomicUnit=on
  PriorityArbitrationCore : MATLAB Function  TreatAsAtomicUnit=on
  ResolvedPressure : Outport
  ResolvedGradient : Outport  Port=2
  ResolvedMode : Outport  Port=3
  ResolvedClipP : Outport  Port=4
  ResolvedClipG : Outport  Port=5
  wires:
  YscValid/1 -> BuildCandidateMatrices/2(YscValid)  "YscValid"
  BuildCandidateMatrices/3(VcGradient) -> PriorityArbitrationCore/3(VcGradient)  "VcGradient"
  BuildCandidateMatrices/2(Pressure) -> PriorityArbitrationCore/2(Pressure)  "Pressure"
  SsmValid/1 -> BuildCandidateMatrices/4(SsmValid)  "SsmValid"
  validatedPressure/1 -> [validatedPressure], PriorityArbitrationCore/6(validatedPressure)  "validatedPressure"
  HpsValid/1 -> BuildCandidateMatrices/5(HpsValid)  "HpsValid"
  PriorityArbitrationCore/2(ResolvedGradient) -> ResolvedGradient/1
  TcValid/1 -> BuildCandidateMatrices/3(TcValid)  "TcValid"
  PriorityArbitrationCore/3(ResolvedMode) -> ResolvedMode/1
  ArbDValid/1 -> BuildCandidateMatrices/1(ArbDValid)  "ArbDValid"
  AbsValid/1 -> BuildCandidateMatrices/6(AbsValid)  "AbsValid"
  BuildCandidateMatrices/1(ActiveMask) -> PriorityArbitrationCore/1(ActiveMask)  "ActiveMask"
  [validatedPressure] -> BuildCandidateMatrices/7(validatedPressure)
  PriorityArbitrationCore/1(ResolvedPressure) -> ResolvedPressure/1
  BuildCandidateMatrices/4(ClipP) -> PriorityArbitrationCore/4(ClipP)
  BuildCandidateMatrices/5(ClipG) -> PriorityArbitrationCore/5(ClipG)
  PriorityArbitrationCore/4(ResolvedClipP) -> ResolvedClipP/1
  PriorityArbitrationCore/5(ResolvedClipG) -> ResolvedClipG/1

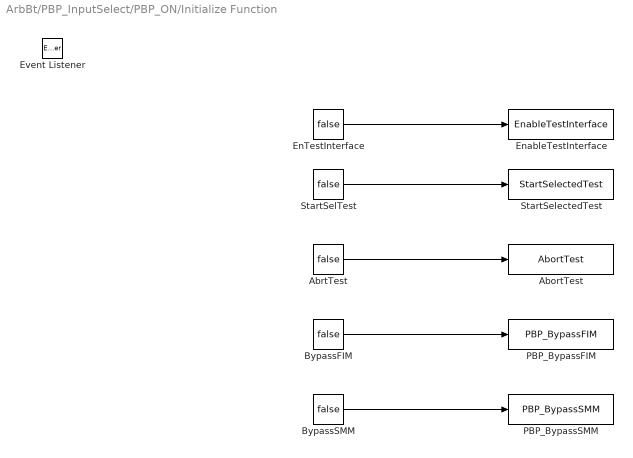
== system ArbBt/PBP_InputSelect/PBP_ON/Initialize Function ==
  AbortTest : DataStoreWrite  DataStoreName=AbortTest  IndexOptions=Index vector (dialog)  Indices=1  OutputSizes=1
  AbrtTest : Constant  Value=false  SampleTime=-1
  BypassFIM : Constant  Value=false  SampleTime=-1
  BypassSMM : Constant  Value=false  SampleTime=-1
  EnTestInterface : Constant  Value=false  SampleTime=-1
  EnableTestInterface : DataStoreWrite  DataStoreName=EnableTestInterface  IndexOptions=Index vector (dialog)  Indices=1  OutputSizes=1
  Event Listener : EventListener  DisableCoverage=on  EventName=reset
  PBP_BypassFIM : DataStoreWrite  DataStoreName=PBP_BypassFIM  IndexOptions=Index vector (dialog)  Indices=1  OutputSizes=1
  PBP_BypassSMM : DataStoreWrite  DataStoreName=PBP_BypassSMM  IndexOptions=Index vector (dialog)  Indices=1  OutputSizes=1
  StartSelTest : Constant  Value=false  SampleTime=-1
  StartSelectedTest : DataStoreWrite  DataStoreName=StartSelectedTest  IndexOptions=Index vector (dialog)  Indices=1  OutputSizes=1
  wires:
  EnTestInterface/1 -> EnableTestInterface/1
  StartSelTest/1 -> StartSelectedTest/1
  AbrtTest/1 -> AbortTest/1
  BypassFIM/1 -> PBP_BypassFIM/1
  BypassSMM/1 -> PBP_BypassSMM/1

== system ArbBt/PBP_InputSelect/PBP_ON/PBP_Control ==
  PBP_StateMachine : Stateflow chart  TreatAsAtomicUnit=on
  PBP_Status : Outport
  PBP_CurrentCycle : Outport  Port=2
  PBP_EntryIndex : Outport  Port=3
  PBP_ActiveRow : Outport  Port=4
  wires:
  PBP_StateMachine/1(PBP_Status) -> PBP_Status/1  "PBP_Status"
  PBP_StateMachine/2(PBP_CurrentCycle) -> PBP_CurrentCycle/1  "PBP_CurrentCycle"
  PBP_StateMachine/3(PBP_EntryIndex) -> PBP_EntryIndex/1  "PBP_EntryIndex"
  PBP_StateMachine/4(PBP_ActiveRow) -> PBP_ActiveRow/1  "PBP_ActiveRow"

== system ArbBt/ArbBt_Arbitrate/ActM_ReleaseVehicleControl/ReleaseWrapper/PBP_OFF ==
  ActM_RelVehCtrl : MATLAB Function  TreatAsAtomicUnit=on

== system ArbBt/ArbBt_Arbitrate/ActM_ReleaseVehicleControl/ReleaseWrapper/PBP_ON ==
  Data Store Read : DataStoreRead  DataStoreName=PBP_BypassSMM  IndexOptions=Index vector (dialog)  Indices=1  OutputSizes=1
  If : If  IfExpression=u1 == 0  ShowElse=off
  ReleaseCall : Subsystem  TreatAsAtomicUnit=on
  wires:
  Data Store Read/1 -> If/1
  If/1 -> ReleaseCall/Action

== system ArbBt/ArbBt_Arbitrate/ArbBt_StateMachine/ActM_Query/PBP_OFF ==
  FiM_Caller : FunctionCaller  FunctionPrototype=FiM_permission = ArbBt_StateMachine.FiM_GetFunctionPermission()  InputArgumentSpecifications=<Enter example>  OutputArgumentSpecifications=boolean(1)  SampleTime=0.005
  Permission : Outport
  wires:
  FiM_Caller/1 -> Permission/1  "FiM_Permission"

== system ArbBt/ArbBt_Arbitrate/ArbBt_StateMachine/ActM_Query/PBP_ON ==
  If : If  IfExpression=u1 == 0
  If Action Subsystem : Subsystem  TreatAsAtomicUnit=on
  If Action Subsystem1 : Subsystem  TreatAsAtomicUnit=on
  Merge : Merge
  PBP_BypassSMM : DataStoreRead  DataStoreName=PBP_BypassSMM  IndexOptions=Index vector (dialog)  Indices=1  OutputSizes=1
  Permission : Outport
  wires:
  If/2 -> If Action Subsystem1/Action
  If/1 -> If Action Subsystem/Action
  PBP_BypassSMM/1 -> If/1
  If Action Subsystem/1(Out1) -> Merge/1
  If Action Subsystem1/1(Out1) -> Merge/2
  Merge/1 -> Permission/1

== system ArbBt/ArbBt_Arbitrate/ArbBt_StateMachine/FiM_Query/PBP_OFF ==
  FiM_Caller : FunctionCaller  FunctionPrototype=FiM_permission = ArbBt_StateMachine.FiM_GetFunctionPermission()  InputArgumentSpecifications=<Enter example>  OutputArgumentSpecifications=boolean(1)  SampleTime=0.005
  Permission : Outport
  wires:
  FiM_Caller/1 -> Permission/1  "FiM_Permission"

== system ArbBt/ArbBt_Arbitrate/ArbBt_StateMachine/FiM_Query/PBP_ON ==
  If : If  IfExpression=u1 == 0
  If Action Subsystem : Subsystem  TreatAsAtomicUnit=on
  If Action Subsystem1 : Subsystem  TreatAsAtomicUnit=on
  Merge : Merge
  PBP_ByPassFIM : DataStoreRead  DataStoreName=PBP_BypassFIM  IndexOptions=Index vector (dialog)  Indices=1  OutputSizes=1
  Permission : Outport
  wires:
  If/2 -> If Action Subsystem1/Action
  If/1 -> If Action Subsystem/Action
  PBP_ByPassFIM/1 -> If/1
  If Action Subsystem/1(Out1) -> Merge/1
  If Action Subsystem1/1(Out1) -> Merge/2
  Merge/1 -> Permission/1

== system ArbBt/ArbBt_Arbitrate/ArbBt_StateMachine/VehCtrlReq_Query/PBP_OFF ==
  FiM_Caller : FunctionCaller  FunctionPrototype=FiM_permission = ArbBt_StateMachine.FiM_GetFunctionPermission()  InputArgumentSpecifications=<Enter example>  OutputArgumentSpecifications=boolean(1)  SampleTime=0.005
  VcReq : Outport
  wires:
  FiM_Caller/1 -> VcReq/1  "FiM_Permission"

== system ArbBt/ArbBt_Arbitrate/ArbBt_StateMachine/VehCtrlReq_Query/PBP_ON ==
  If : If  IfExpression=u1 == 0
  If Action Subsystem : Subsystem  TreatAsAtomicUnit=on
  If Action Subsystem1 : Subsystem  TreatAsAtomicUnit=on
  Merge : Merge
  PBP_BypassSMM : DataStoreRead  DataStoreName=PBP_BypassSMM  IndexOptions=Index vector (dialog)  Indices=1  OutputSizes=1
  VcReq : Outport
  wires:
  If/2 -> If Action Subsystem1/Action
  If/1 -> If Action Subsystem/Action
  PBP_BypassSMM/1 -> If/1
  If Action Subsystem/1(Out1) -> Merge/1
  If Action Subsystem1/1(Out1) -> Merge/2
  Merge/1 -> VcReq/1

== system ArbBt/ArbBt_Arbitrate/ActM_ReleaseVehicleControl/ReleaseWrapper/PBP_ON/ReleaseCall ==
  note: Place ActMVehicleControlRelease here. Skipped when PBP_BypassSMM = True
  Action Port : ActionPort  ActionPortLabel=if(u1 == 0)
  ActM_RelVehCtrl : MATLAB Function  TreatAsAtomicUnit=on

== system ArbBt/ArbBt_Arbitrate/ArbBt_StateMachine/ActM_Query/PBP_ON/If Action Subsystem ==
  Action Port : ActionPort  ActionPortLabel=if(u1 == 0)
  ActM_Caller : FunctionCaller  FunctionPrototype=ActM_ArbPermission = ArbBt_StateMachine.ActM_GetArbitratorPermission()  InputArgumentSpecifications=<Enter example>  OutputArgumentSpecifications=boolean(1)  SampleTime=0.005
  Out1 : Outport
  wires:
  ActM_Caller/1 -> Out1/1  "ActM_ArbPermission"

== system ArbBt/ArbBt_Arbitrate/ArbBt_StateMachine/ActM_Query/PBP_ON/If Action Subsystem1 ==
  Action Port : ActionPort  ActionPortLabel=else
  Constant : Constant  Value=true  OutDataTypeStr=boolean  SampleTime=-1
  Out1 : Outport
  wires:
  Constant/1 -> Out1/1

== system ArbBt/ArbBt_Arbitrate/ArbBt_StateMachine/FiM_Query/PBP_ON/If Action Subsystem ==
  Action Port : ActionPort  ActionPortLabel=if(u1 == 0)
  FiM_Caller : FunctionCaller  FunctionPrototype=FiM_permission = ArbBt_StateMachine.FiM_GetFunctionPermission()  InputArgumentSpecifications=<Enter example>  OutputArgumentSpecifications=boolean(1)  SampleTime=0.005
  Out1 : Outport
  wires:
  FiM_Caller/1 -> Out1/1  "FiM_Permission"

== system ArbBt/ArbBt_Arbitrate/ArbBt_StateMachine/FiM_Query/PBP_ON/If Action Subsystem1 ==
  Action Port : ActionPort  ActionPortLabel=else
  Constant : Constant  Value=true  OutDataTypeStr=boolean  SampleTime=-1
  Out1 : Outport
  wires:
  Constant/1 -> Out1/1

== system ArbBt/ArbBt_Arbitrate/ArbBt_StateMachine/VehCtrlReq_Query/PBP_ON/If Action Subsystem ==
  Action Port : ActionPort  ActionPortLabel=if(u1 == 0)
  VehCtrlReqCaller : FunctionCaller  FunctionPrototype=ActM_ReqVehControl_Granted = ArbBt_StateMachine.ActM_RequestVehicleControl()  InputArgumentSpecifications=<Enter example>  OutputArgumentSpecifications=boolean(1)  SampleTime=0.005
  Out1 : Outport
  wires:
  VehCtrlReqCaller/1 -> Out1/1  "ActM_ReqVehControl_Granted"

== system ArbBt/ArbBt_Arbitrate/ArbBt_StateMachine/VehCtrlReq_Query/PBP_ON/If Action Subsystem1 ==
  Action Port : ActionPort  ActionPortLabel=else
  Constant : Constant  Value=true  OutDataTypeStr=boolean  SampleTime=-1
  Out1 : Outport
  wires:
  Constant/1 -> Out1/1

== matlab function ArbBt/ArbBt_Validate/Validate_HpsRequest ==
  data: VcRequestBus input Bus: Bus_VcRequest size=1; ValidatedVcRequestBus output Bus: ValidatedVcRequestBus size=1; ArbBt_PressureInactive parameter single size=1; ArbBt_GradientInactive parameter single size=1; ArbBt_PressureMin parameter single size=1; ArbBt_PressureMax parameter single size=1; ArbBt_GradientMin parameter single size=1; ArbBt_GradientMax parameter single size=1; CLIP_LOW_P parameter single; CLIP_HIGH_P parameter single; CLIP_LOW_G parameter single; CLIP_HIGH_G parameter single
function ValidatedVcRequestBus = ValidateVcRequest( ...
    VcRequestBus, ...
    ArbBt_PressureInactive, ArbBt_GradientInactive, ...
    ArbBt_PressureMin, ArbBt_PressureMax, ...
    ArbBt_GradientMin, ArbBt_GradientMax, ...
    CLIP_LOW_P, CLIP_HIGH_P, CLIP_LOW_G, CLIP_HIGH_G)

% FUNCTION NAME:
%   ValidateVcRequest
%
% DESCRIPTION:
%   Validates the vehicle control request by checking pressure and8
%   gradient values against the configured inactive, minimum, clipping and
%   maximum limits.
%
%   Requirement Reference:
%   Section 11.2, REQ_ASW_ARB_BT_SW_013-017
%
% INPUT:
%   VcRequestBus - Vehicle control request bus.
%   ArbBt_PressureInactive - Inactive pressure reference value.
%   ArbBt_GradientInactive - Inactive gradient reference value.
%   ArbBt_PressureMin - Minimum allowed invalid pressure value.
%   ArbBt_PressureMax - Maximum allowed invalid pressure value.
%   CLIP_LOW_P - Minimum clipping pressure value.
%   CLIP_HIGH_P - Maximum clipping pressure value.
%   ArbBt_GradientMin - Minimum allowed invalid gradient value.
%   ArbBt_GradientMax - Maximum allowed invalid gradient value.
%   CLIP_LOW_G - Minimum clipping gradient value.
%   CLIP_HIGH_G - Maximum clipping gradient value.
% OUTPUT:
%   ValidatedVcRequestBus - Validated vehicle control request output bus.

% Constants
PressureTol = single(0.001);
GradientTol = single(0.001);
%% Wheel Indices
firstWheel = int32(1);
lastWheel  = int32(4);
 
% Initialize

ValidatedVcRequestBus = struct( ...
    'Valid',        false, ...
    'Pressure',     VcRequestBus.Pressure, ...
    'VcGradient',   VcRequestBus.VcGradient, ...
    'Requested',    VcRequestBus.Requested, ...
    'WheelValid',   false(1, 4), ...
    'ClipPressure', false(1, 4), ...
    'ClipGradient', false(1, 4));
%% Validate Wheel Requests
for w = firstWheel:lastWheel
    req = VcRequestBus.Requested(w);
    noRequest     = req == ArbBtVcRequest.NO_REQUEST;
    activeRequest = (req == ArbBtVcRequest.REQUEST) ||...
        (req == ArbBtVcRequest.REQUEST_BPF);
 %% No Request
    if noRequest
        inactiveValuesOk = ...
            abs(VcRequestBus.Pressure(w)   - ArbBt_PressureInactive) <= ...
            PressureTol && ...
            abs(VcRequestBus.VcGradient(w) - ArbBt_GradientInactive) <= ...
            GradientTol;
        if inactiveValuesOk
            ValidatedVcRequestBus.WheelValid(w) = true;
	else
	    % Inactive pressure or gradient is outside
            % allowed tolerance.
        end
 %% Active Request
    elseif activeRequest
        rawPressure = VcRequestBus.Pressure(w);
        rawGradient = VcRequestBus.VcGradient(w);
 
        % Stage 1: outside the physical range = invalid, no clipping, 
        % no flag.
        requestValuesOk = ...
            rawPressure >= ArbBt_PressureMin && rawPressure <=...
            ArbBt_PressureMax && ...
            rawGradient >= ArbBt_GradientMin && rawGradient <=...
            ArbBt_GradientMax;
 %% Validate Pressure and Gradient
        if requestValuesOk
            % Stage 2: clip to the tighter band and flag only 
            % if the value changed.
            ValidatedVcRequestBus.Pressure(w)     =...
                min(max(rawPressure, CLIP_LOW_P), CLIP_HIGH_P);
            ValidatedVcRequestBus.VcGradient(w)   =...
                min(max(rawGradient, CLIP_LOW_G), CLIP_HIGH_G);
            ValidatedVcRequestBus.ClipPressure(w) =...
                (rawPressure < CLIP_LOW_P) || (rawPressure > CLIP_HIGH_P);
            ValidatedVcRequestBus.ClipGradient(w) =....
                (rawGradient < CLIP_LOW_G) || (rawGradient > CLIP_HIGH_G);
            ValidatedVcRequestBus.WheelValid(w)   = true;
	else
	   % Requested pressure or gradient is outside range
        end
    else
	% Unsupported request value.
        % Retain initialized invalid output.
    end
end
% Overall Validity
ValidatedVcRequestBus.Valid = all(ValidatedVcRequestBus.WheelValid);
end
